simulink subsystem "tDMSquared_Error"  (R2024b)
settings: Solver=VariableStepAuto  StartTime=0.0  StopTime=10.0  RelTol=1e-3
model mask{messageText='This is a tDMSquared message.', T_s=1e-4, stopSim=on}
  mask prompts: messageText "Message Text:"; T_s "Sample Time [s]:"; stopSim "Stop simulation after creating error message"
libraries: simulink x2
settings Model: Creator=winkens  LastModifiedBy=k.kocaogullar
settings SolverCC: AlgebraicLoopSolver=TrustRegion
settings OptimizationCC: ReuseModelBlockBuffer=off
settings DebuggingCC: UnconnectedInputMsg=warning  UnconnectedOutputMsg=warning  UnconnectedLineMsg=warning
settings ModelReferenceCC: EnableRefExpFcnMdlSchedulingChecks=on
settings RTWCC: GPUComputeCapability=3.5  DLArmComputeVersion=19.05

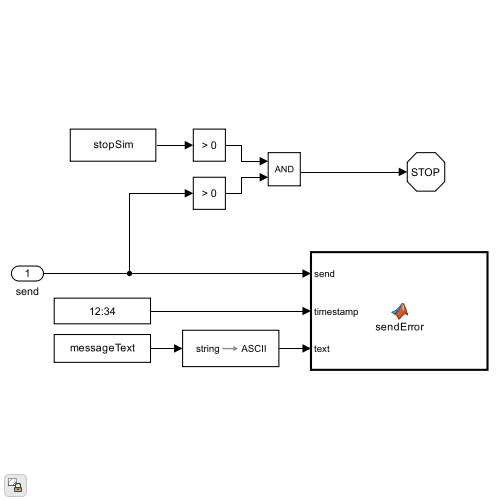
[thumbnail: Simulink's stored preview of the top-level diagram]
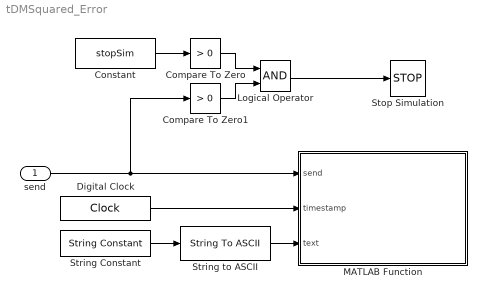
== system tDMSquared_Error ==
  send : Inport
  Compare To Zero : simulink/Logic and Bit Operations/Compare To Zero  relop=>  OutDataTypeStr=boolean
  Compare To Zero1 : simulink/Logic and Bit Operations/Compare To Zero  relop=>  OutDataTypeStr=boolean
  Constant : Constant  Value=stopSim
  Digital Clock : DigitalClock  SampleTime=T_s
  Logical Operator : Logic  AllPortsSameDT=off  OutDataTypeStr=boolean
  MATLAB Function : MATLAB Function  TreatAsAtomicUnit=on
  Stop Simulation : Stop
  String Constant : StringConstant  String=messageText  OutDataTypeStr=stringtype(300)
  String to ASCII : StringToASCII  OutputVectorSize=300
  wires:
  send/1 -> MATLAB Function/1(send), Compare To Zero1/1
  String Constant/1 -> String to ASCII/1
  Digital Clock/1 -> MATLAB Function/2(timestamp)
  String to ASCII/1 -> MATLAB Function/3(text)
  Constant/1 -> Compare To Zero/1
  Compare To Zero/1 -> Logical Operator/1
  Compare To Zero1/1 -> Logical Operator/2
  Logical Operator/1 -> Stop Simulation/1

== matlab function tDMSquared_Error/MATLAB Function ==
  data: send input; timestamp input; text input
function sendError(send,timestamp, text)
   coder.extrinsic('sldiagviewer.reportError');
   coder.extrinsic('gcb');
   %Usage of feval necessary to force usage of Matlab interpreter
   coder.extrinsic('feval');
   if send  
       blockName = gcb;
       message = feval('create_tdm2_Message','error',timestamp,blockName,text);
       sldiagviewer.reportError(message);
    end
end
